simulink library "WECSim_Lib_Body_Elements"  (R2020b)
settings: Solver=VariableStepAuto  StartTime=0.0  StopTime=10.0  RelTol=1e-3
undefined symbols (not defined in the file or in its folder): body, simu, waves, X, Y, Z
libraries: nesl_utility x22, sm_lib x16, $bdroot x9, vrlib x3
(part 1 of 5)
settings Model: Creator=kmruehl  LastModifiedBy=rsaucie
settings ConfigComp: CovBoundaryAbsTol=1.0e-5

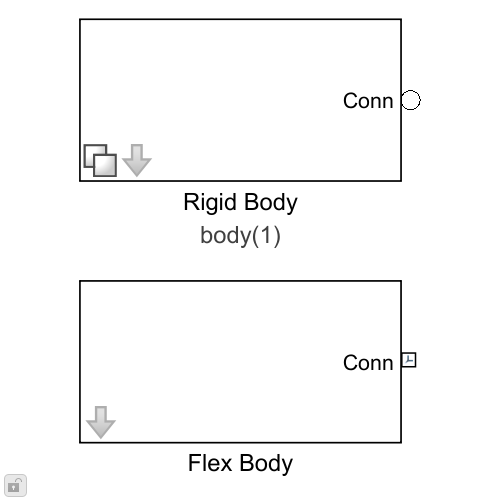
[thumbnail: Simulink's stored preview of the top-level diagram]
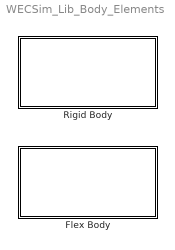
== system WECSim_Lib_Body_Elements ==
  Flex Body : Subsystem  VariantControl=(default)  mask(Flex Body){body=body(1)}
      mask prompts: body "Body Number:"
      mask help:
      | A Flex Body may contain generalized body modes that account for various bending, shear or other deformation modes. The BEM output must contain data for these additional DOFs.
      |
      | The variable name input below must be 'body(i)' where i=1,2,...
      | body(i) must be defined in the input file with the following fields:
      |
      |     .flexHydroBody = 1 (required)
      |             Float.
      |             Flag that creates a flex body. Set equal to 1 if the BEM data contains more than 6 degrees of freedom.
      |     .filename (required)
      |             String.
      |             The file path specifying the .h5 file for the body.
      |     .mass (required)
      |             Float or string.
      |             The translational interia or mass of the body in kg. If a string, the value must be 'equilibrium'. Default = [ ]
      |     .momOfIntertia (required)
      |             3x1 vector [Ixx Iyy Izz].
      |             Rotational intertia of the body in kg*m^2. Default = [ ]
      |     .geometryFile (optional)
      |             String
      |             Path to the geometry file of the body (.stl). Required for nonlinear hydrodynamics or visualization. Default = [ ]
      mask init:
      | if exist('body','var')
      |     % geometry file name
      |     h=[gcb '/Structure/Body Properties'];
      |     geomFile=body.geometryFile;
      |     set_param(h,'ExtGeomFileName',geomFile);
      |     geomType='STL';
      |     % split version e.g. '9.10.0.16028 (R2021a)' into 9, 10, 0, NaN.
      |     % cannot compare str2double('9.10') because it becomes '9.1' 
      |     ver=split(version,'.');
      |     ver=str2double(ver(1:3));
      |     if ver(1) < 9 || (ver(1) == 9 && ver(2) < 6)
      |        set_param(h,'ExtGeomFileType',geomType);
      |     end
      |     % toWorkSpace: outputs
      |     h=[gcb '/To Workspace'];
      |     responseName=['body' num2str(body.number) '_out'];
      |     set_param(h,'VariableName',responseName);
      |     % toWorkSpace: hydrostatic pressures
      |     h=[gcb '/Hydrostatic Restoring Force Calculation/Hydrostatic Restoring Force Calculation/Linear and Nonlinear Restoring Force Variant Subsystem/Nonlinear Hydrostatic Restoring Force/To Workspace1'];
      |     responseName=['body' num2str(body.number) '_hspressure_out'];
      |     set_param(h,'VariableName',responseName); 
      |     % toWorkSpace: wave pressures (nonlinear Froude-Krylov)
      |     h=[gcb '/Wave Diffraction and Excitation Force Calculation/Wave Diffraction and Excitation Force Calculation/Nonlinear FK Force Variant Subsystem/With Nonlinear FroudeKrylov Force/To Workspace'];
      |     responseName=['body' num2str(body.number) '_wavenonlinearpressure_out'];
      |     set_param(h,'VariableName',responseName);
      |     % toWorkSpace: wave pressures (linear Froude-Krylov)
      |     h=[gcb '/Wave Diffraction and Excitation Force Calculation/Wave Diffraction and Excitation Force Calculation/Nonlinear FK Force Variant Subsystem/With Nonlinear FroudeKrylov Force/To Workspace1'];
      |     responseName=['body' num2str(body.number) '_wavelinearpressure_out'];
      |     set_param(h,'VariableName',responseName);
      |     % position: GoTo 
      |     h=[gcb '/Goto'];
      |     responseName=['disp' num2str(body.number)];
      |     set_param(h,'GotoTag',responseName);
      |     % position: From
      |     h=[gcb '/From'];
      |     responseName=['disp' num2str(body.number)];
      |     set_param(h,'GotoTag',responseName);
      |     % velocity: GoTo 
      |     h=[gcb '/Goto1'];
      |     responseName=['vel' num2str(body.number)];
      |     set_param(h,'GotoTag',responseName);
      |     % velocity: From 
      |     h=[gcb '/From1'];
      |     responseName=['vel' num2str(body.number)];
      |     set_param(h,'GotoTag',responseName);
      |     % acceleration: GoTo 
      |     h=[gcb '/Goto2'];
      |     responseName=['acc' num2str(body.number)];
      |     set_param(h,'GotoTag',responseName);
      |     % acceleration: From 
      |     h=[gcb '/From2'];
      |     responseName=['acc' num2str(body.number)];
      |     set_param(h,'GotoTag',responseName);
      |     %% Variable Hydro:
      |     % Variant subsystem
      |     h = [gcb '/Variable Hydrodynamics Control/Variable Hydrodynamics Subsystem'];
      |     responseName = ['sv_b' num2str(body.number) '_variableHydro'];
      |     set_param(h,'VariantControl',responseName);
      |     % body_hydroForceIndex To Workspace tags
      |     h=[gcb '/Variable Hydrodynamics Control/Variable Hydrodynamics Subsystem/variableHydro/To Workspace'];
      |     responseName=['body' num2str(body.number) '_hydroForceIndex'];
      |     set_param(h,'VariableName',responseName); 
      |     % body_hydroForceIndex From tags
      |     h=[gcb '/Variable Hydrodynamics Control/Variable Hydrodynamics Subsystem/variableHydro/From'];
      |     responseName=['body' num2str(body.number) '_hydroForceIndex'];
      |     set_param(h,'GotoTag',responseName);
      |     % body_hydroForce GoTo
      |     h=[gcb '/Variable Hydrodynamics Control/Goto'];
      |     responseName=['body' num2str(body.number) '_hydroForce'];
      |     set_param(h,'GotoTag',responseName);
      |     % body_hydroForce From tags
      |     h=[gcb '/Wave Diffraction and Excitation Force Calculation/Wave Diffraction and Excitation Force Calculation/From'];
      |     responseName=['body' num2str(body.number) '_hydroForce'];
      |     set_param(h,'GotoTag',responseName);
      |     h=[gcb '/Wave Radiation Forces Calculation/Wave Radiation Forces Calculation/From'];
      |     responseName=['body' num2str(body.number) '_hydroForce'];
      |     set_param(h,'GotoTag',responseName);
      |     h=[gcb '/Wave Radiation Forces Calculation/Wave Radiation Forces Calculation/SS CI and Constant-Damping-CoeVariant Subsystem/Constant Coefficients/From'];
      |     responseName=['body' num2str(body.number) '_hydroForce'];
      |     set_param(h,'GotoTag',responseName);
      |     h=[gcb '/Wave Radiation Forces Calculation/Wave Radiation Forces Calculation/SS CI and Constant-Damping-CoeVariant Subsystem/Convolution Integral Calculation/Convolution Variant Subsystem/Convolution Integral Calculation/From'];
      |     responseName=['body' num2str(body.number) '_hydroForce'];
      |     set_param(h,'GotoTag',responseName);
      |     h=[gcb '/Wave Radiation Forces Calculation/Wave Radiation Forces Calculation/SS CI and Constant-Damping-CoeVariant Subsystem/Convolution Integral Calculation/Convolution Variant Subsystem/Convolution Integral Surface Calculation/From'];
      |     responseName=['body' num2str(body.number) '_hydroForce'];
      |     set_param(h,'GotoTag',responseName);
      |     h=[gcb '/Hydrostatic Restoring Force Calculation/Hydrostatic Restoring Force Calculation/Linear and Nonlinear Restoring Force Variant Subsystem/Linear Hydrostatic Restoring Force/From'];
      |     responseName=['body' num2str(body.number) '_hydroForce'];
      |     set_param(h,'GotoTag',responseName);
      |     h=[gcb '/Hydrostatic Restoring Force Calculation/Hydrostatic Restoring Force Calculation/Linear and Nonlinear Restoring Force Variant Subsystem/Nonlinear Hydrostatic Restoring Force/From'];
      |     responseName=['body' num2str(body.number) '_hydroForce'];
      |     set_param(h,'GotoTag',responseName);
      |     h=[gcb '/Hydrostatic Restoring Force Calculation/Hydrostatic Restoring Force Calculation/From'];
      |     responseName=['body' num2str(body.number) '_hydroForce'];
      |     set_param(h,'GotoTag',responseName);
      |     h=[gcb '/Morrison Element and Viscous Damping Force Calculation/From'];
      |     responseName=['body' num2str(body.number) '_hydroForce'];
      |     set_param(h,'GotoTag',responseName);
      |     h=[gcb '/Additional Linear Damping Force Calculation/From'];
      |     responseName=['body' num2str(body.number) '_hydroForce'];
      |     set_param(h,'GotoTag',responseName);
      |     h=[gcb '/FlexibleBody/From'];
      |     responseName=['body' num2str(body.number) '_hydroForce'];
      |     set_param(h,'GotoTag',responseName);
      |     % Update body.hydroForce constant data type
      |     h=[gcb '/Variable Hydrodynamics Control/Constant'];
      |     busName=['Bus: bus_body' num2str(body.number) '_hydroForce'];
      |     set_param(h,'OutDataTypeStr',busName);
      |     %%
      |     % Flex Body Morison Element: Off
      |     h = [gcb '/Morrison Element and Viscous Damping Force Calculation/Morison Element and Viscous Damping Force Calculation/Morison Element Variant Subsystem/Morison Element Off'];
      |     responseName = ['sv_b' num2str(body.number) '_MEOff'];
      |     set_param(h,'VariantControl',responseName);
      |     %%
      |     % Flex Body Morison Element: On
      |     h = [gcb '/Morrison Element and Viscous Damping Force Calculation/Morison Element and Viscous Damping Force Calculation/Morison Element Variant Subsystem/Morison Element On'];
      |     responseName = ['sv_b' num2str(body.number) '_MEOn'];
      |     set_param(h,'VariantControl',responseName);
      |     %%
      |     % Flex Body Nonlinear FroudeKrylov Force: Off
      |     h = [gcb '/Wave Diffraction and Excitation Force Calculation/Wave Diffraction and Excitation Force Calculation/Nonlinear FK Force Variant Subsystem/No Nonlinear FroudeKrylov Force'];
      |     responseName = ['sv_b' num2str(body.number) '_linearHydro'];
      |     set_param(h,'VariantControl',responseName);
      |     %%
      |     % Flex Body Nonlinear FroudeKrylov Force: On
      |     h = [gcb '/Wave Diffraction and Excitation Force Calculation/Wave Diffraction and Excitation Force Calculation/Nonlinear FK Force Variant Subsystem/With Nonlinear FroudeKrylov Force'];
      |     responseName = ['sv_b' num2str(body.number) '_nonlinearHydro'];
      |     set_param(h,'VariantControl',responseName);
      |     %%
      |     % Flex Body Nonlinear Restoring: Off
      |     h = [gcb '/Hydrostatic Restoring Force Calculation/Hydrostatic Restoring Force Calculation/Linear and Nonlinear Restoring Force Variant Subsystem/Linear Hydrostatic Restoring Force'];
      |     responseName = ['sv_b' num2str(body.number) '_linearHydro'];
      |     set_param(h,'VariantControl',responseName);
      |     %%
      |     % Flex Body Nonlinear Restoring: On
      |     h = [gcb '/Hydrostatic Restoring Force Calculation/Hydrostatic Restoring Force Calculation/Linear and Nonlinear Restoring Force Variant Subsystem/Nonlinear Hydrostatic Restoring Force'];
      |     responseName = ['sv_b' num2str(body.number) '_nonlinearHydro'];
      |     set_param(h,'VariantControl',responseName);
      |     %%
      |     % Flex Body Nonlinear FroudeKrylov or Restoring: Instantaneous Free Surface
      |     h = [gcb '/Nonlinear Wave Elevation/Linear or Instantaneous Free Surface/Instantaneous Water Free Surface'];
      |     responseName = ['sv_b' num2str(body.number) '_instFS'];
      |     set_param(h,'VariantControl',responseName);
      |     %%
      |     % Flex Body Nonlinear FroudeKrylov or Restoring: Mean Free Surface
      |     h = [gcb '/Nonlinear Wave Elevation/Linear or Instantaneous Free Surface/Mean Water Free Surface'];
      |     responseName = ['sv_b' num2str(body.number) '_meanFS'];
      |     set_param(h,'VariantControl',responseName);
      |     %%
      | end
      mask Help:
      | A Flex Body may contain generalized body modes that account for various bending, shear or other deformation modes. The BEM output must contain data for these additional DOFs.
      | 
      | The variable name input below must be 'body(i)' where i=1,2,...
      | body(i) must be defined in the input file with the following fields:
      | 
      |     .flexHydroBody = 1 (required)
      |             Float.
      |             Flag that creates a flex body. Set equal to 1 if the BEM data contains more than 6 degrees of freedom.
      |     .filename (required)
      |             String.
      |             The file path specifying the .h5 file for the body.
      |     .mass (required)
      |             Float or string.
      |             The translational interia or mass of the body in kg. If a string, the value must be 'equilibrium'. Default = [ ]
      |     .momOfIntertia (required)
      |             3x1 vector [Ixx Iyy Izz].
      |             Rotational intertia of the body in kg*m^2. Default = [ ]
      |     .geometryFile (optional)
      |             String
      |             Path to the geometry file of the body (.stl). Required for nonlinear hydrodynamics or visualization. Default = [ ]
  Rigid Body : Subsystem  Variant=on  AllowZeroVariantControls=on  mask(Rigid Body){body=body(1)}
      mask prompts: body "Body Number:"
      mask help:
      | A rigid body has no generalized body modes. It can be a standard hydrodynamic body, a drag body, or a non-hydrodynamic body.
      |
      | The variable name input below must be 'body(i)' where i=1,2,...
      | body(i) must be defined in the input file with the fields appropriate to each variant.
      mask init:
      | if exist('body','var')
      |     %%
      |     % Hydro Body
      |     h = [gcb '/Hydrodynamic Body'];
      |     responseName = ['sv_b' num2str(body.number) '_hydroBody'];
      |     set_param(h,'VariantControl',responseName);
      |     %%
      |     % Hydro Body Morison Element: Off
      |     h = [gcb '/Hydrodynamic Body/Morison Element and Viscous Damping Force Calculation/Morison Element Variant Subsystem/Morison Element Off'];
      |     responseName = ['sv_b' num2str(body.number) '_MEOff'];
      |     set_param(h,'VariantControl',responseName);
      |     %%
      |     % Hydro Body Morison Element: On
      |     h = [gcb '/Hydrodynamic Body/Morison Element and Viscous Damping Force Calculation/Morison Element Variant Subsystem/Morison Element On'];
      |     responseName = ['sv_b' num2str(body.number) '_MEOn'];
      |     set_param(h,'VariantControl',responseName);
      |     %%
      |     % Hydro Body Nonlinear Froude Krylov Force: Off
      |     h = [gcb '/Hydrodynamic Body/Wave Diffraction and Excitation Force Calculation/Nonlinear FK Force Variant Subsystem/No Nonlinear FroudeKrylov Force'];
      |     responseName = ['sv_b' num2str(body.number) '_linearHydro'];
      |     set_param(h,'VariantControl',responseName);
      |     %%
      |     % Hydro Body Nonlinear Froude Krylov Force: On
      |     h = [gcb '/Hydrodynamic Body/Wave Diffraction and Excitation Force Calculation/Nonlinear FK Force Variant Subsystem/With Nonlinear FroudeKrylov Force'];
      |     responseName = ['sv_b' num2str(body.number) '_nonlinearHydro'];
      |     set_param(h,'VariantControl',responseName);
      |     %%
      |     % Hydro Body Nonlinear Restoring: Off
      |     h = [gcb '/Hydrodynamic Body/Hydrostatic Restoring Force Calculation/Linear and Nonlinear Restoring Force Variant Subsystem/Linear Hydrostatic Restoring Force'];
      |     responseName = ['sv_b' num2str(body.number) '_linearHydro'];
      |     set_param(h,'VariantControl',responseName);
      |     %%
      |     % Hydro Body Nonlinear Restoring: On
      |     h = [gcb '/Hydrodynamic Body/Hydrostatic Restoring Force Calculation/Linear and Nonlinear Restoring Force Variant Subsystem/Nonlinear Hydrostatic Restoring Force'];
      |     responseName = ['sv_b' num2str(body.number) '_nonlinearHydro'];
      |     set_param(h,'VariantControl',responseName);
      |     %%
      |     % Hydro Body Regular Excitation Passive Yaw: Off
      |     h = [gcb '/Hydrodynamic Body/Wave Diffraction and Excitation Force Calculation/Linear Wave Excitation Force Variant Subsystem/Regular Wave ' newline 'Excitation Force'];
      |     responseName = ['sv_regularWaves_b' num2str(body.number)];
      |     set_param(h,'VariantControl',responseName);
      |     %%
      |     % Hydro Body Regular Excitation Passive Yaw: On
      |     h = [gcb '/Hydrodynamic Body/Wave Diffraction and Excitation Force Calculation/Linear Wave Excitation Force Variant Subsystem/Regular Wave ' newline 'NonLinear Yaw'];
      |     responseName = ['sv_regularWavesYaw_b' num2str(body.number)];
      |     set_param(h,'VariantControl',responseName);
      |     %%    
      |     % Hydro Body Irregular Excitation Passive Yaw: Off
      |     h = [gcb '/Hydrodynamic Body/Wave Diffraction and Excitation Force Calculation/Linear Wave Excitation Force Variant Subsystem/Irregular Wave ' newline 'Excitation Force'];
      |     responseName = ['sv_irregularWaves_b' num2str(body.number)];
      |     set_param(h,'VariantControl',responseName);
      |     %%
      |     % Hydro Body Irregular Excitation Passive Yaw: On
      |     h = [gcb '/Hydrodynamic Body/Wave Diffraction and Excitation Force Calculation/Linear Wave Excitation Force Variant Subsystem/Irregular Wave ' newline 'NonLinearYaw'];
      |     responseName = ['sv_irregularWavesYaw_b' num2str(body.number)];
      |     set_param(h,'VariantControl',responseName);
      |     %%
      |     % Hydro Body Nonlinear Froude Krylov or Restoring: Instantaneous Free Surface
      |     h = [gcb '/Hydrodynamic Body/Nonlinear Wave Elevation/Linear or Instantaneous Free Surface/Instantaneous Water Free Surface'];
      |     responseName = ['sv_b' num2str(body.number) '_instFS'];
      |     set_param(h,'VariantControl',responseName);
      |     %%
      |     % Hydro Body Nonlinear Froude Krylov or Restoring: Mean Free Surface
      |     h = [gcb '/Hydrodynamic Body/Nonlinear Wave Elevation/Linear or Instantaneous Free Surface/Mean Water Free Surface'];
      |     responseName = ['sv_b' num2str(body.number) '_meanFS'];
      |     set_param(h,'VariantControl',responseName);
      |     %% Variable hydro on/off
      |     % Variable hydro control - variable hydro off
      |     h = [gcb '/Hydrodynamic Body/Variable Hydrodynamics Control/Variable Hydrodynamics Subsystem/noVariableHydro'];
      |     responseName = ['sv_b' num2str(body.number) '_noVariableHydro'];
      |     set_param(h,'VariantControl',responseName);
      |     % Variable hydro control - variable hydro on
      |     h = [gcb '/Hydrodynamic Body/Variable Hydrodynamics Control/Variable Hydrodynamics Subsystem/variableHydro'];
      |     responseName = ['sv_b' num2str(body.number) '_variableHydro'];
      |     set_param(h,'VariantControl',responseName);
      |     % CIC - variable hydro off
      |     h = [gcb '/Hydrodynamic Body/Wave Radiation Forces Calculation/SS CI and Constant-Damping-CoeVariant Subsystem/Convolution Integral Calculation/Convolution Variant Subsystem/Convolution Integral Calculation'];
      |     responseName = ['sv_b' num2str(body.number) '_noVariableHydro'];
      |     set_param(h,'VariantControl',responseName);
      |     % CIC - variable hydro on
      |     h = [gcb '/Hydrodynamic Body/Wave Radiation Forces Calculation/SS CI and Constant-Damping-CoeVariant Subsystem/Convolution Integral Calculation/Convolution Variant Subsystem/Convolution Integral Surface Calculation'];
      |     responseName = ['sv_b' num2str(body.number) '_variableHydro'];
      |     set_param(h,'VariantControl',responseName);
      |     %%
      |     % Drag Body
      |     h = [gcb '/Drag Body'];
      |     responseName = ['sv_b' num2str(body.number) '_dragBody'];
      |     set_param(h,'VariantControl',responseName);
      |     %%
      |     % Drag Body Morison Element: Off
      |     h = [gcb '/Drag Body/Morison Element and Viscous Damping Force Calculation/Morison Element Variant Subsystem/Morison Element Off'];
      |     responseName = ['sv_b' num2str(body.number) '_MEOff'];
      |     set_param(h,'VariantControl',responseName);
      |     %%
      |     % Drag Body Morison Element: On
      |     h = [gcb '/Drag Body/Morison Element and Viscous Damping Force Calculation/Morison Element Variant Subsystem/Morison Element On'];
      |     responseName = ['sv_b' num2str(body.number) '_MEOn'];
      |     set_param(h,'VariantControl',responseName);
      |     %% 
      |     % Hydro Body QTF: Off
      |     h = [gcb '/Hydrodynamic Body/Wave Diffraction and Excitation Force Calculation/Second Order Excitation Force Variant Subsystem/No Second Order Excitation Force'];
      |     responseName = ['sv_b' num2str(body.number) '_noSecondOrderExt'];
      |     set_param(h,'VariantControl',responseName);
      |     %%
      |     % Hydro Body QTF: On
      |     h = [gcb '/Hydrodynamic Body/Wave Diffraction and Excitation Force Calculation/Second Order Excitation Force Variant Subsystem/With Second Order Excitation Force'];
      |     responseName = ['sv_b' num2str(body.number) '_secondOrderExt'];
      |     set_param(h,'VariantControl',responseName);
      |     %%
      |     % Set zero active variant controls to prevent label issue
      |     set_param(gcb,'AllowZeroVariantControls','on');
      | end
      | clear bc h geomFile responseName
      settings: AttributesFormatString=%<body>
      mask Help:
      | A rigid body has no generalized body modes. It can be a standard hydrodynamic body, a drag body, or a non-hydrodynamic body.
      | 
      | The variable name input below must be 'body(i)' where i=1,2,...
      | body(i) must be defined in the input file with the fields appropriate to each variant.

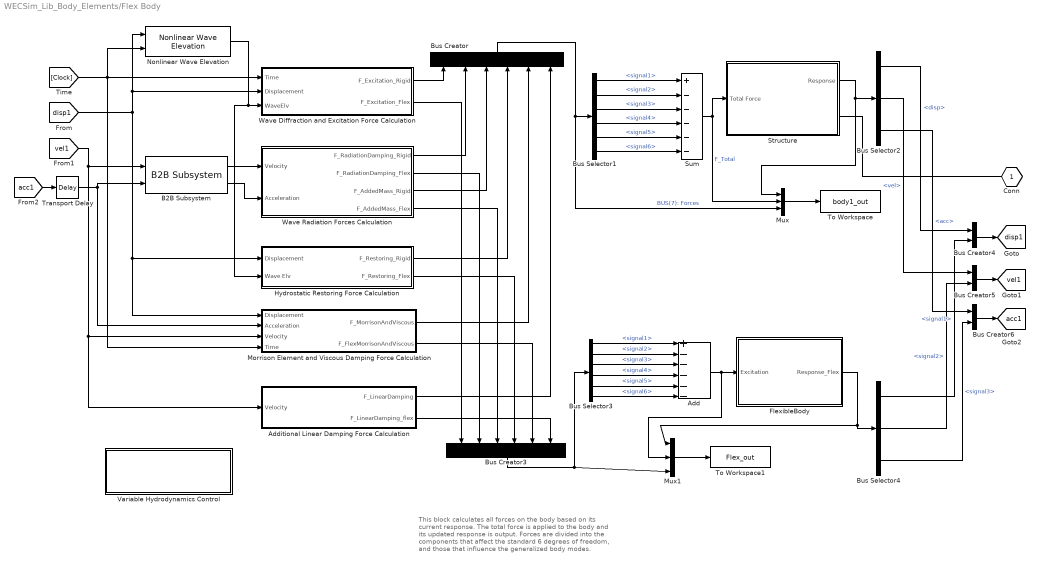
== system WECSim_Lib_Body_Elements/Flex Body ==
  note: This block calculates all forces on the body based on its current response. The total force is applied to the body and its updated response is output.
      |
      | Forces are divided into the components that affect the standard 6 degrees of freedom, and those that influence the generalized body modes.
  Add : Sum  Inputs=+-----
  Additional Linear Damping Force Calculation : Subsystem
  B2B Subsystem : $bdroot/Rigid Body/Hydrodynamic Body/B2B Subsystem  SystemSampleTime=-1  VariantActivationTime=update diagram  EmptyChoice=off  PassThrough=off  PassThroughVariantControl=(default)  EmptyChoiceVariantControl=(default)  Latency=0  AutoFrameSizeCalculation=off
  Bus Creator : BusCreator  Inputs=6
  Bus Creator3 : BusCreator  Inputs=6
  Bus Creator4 : BusCreator  Inputs=2
  Bus Creator5 : BusCreator  Inputs=2
  Bus Creator6 : BusCreator  Inputs=2
  Bus Selector1 : BusSelector  OutputSignals=signal1,signal2,signal3,signal4,signal5,signal6
  Bus Selector2 : BusSelector  OutputSignals=disp,vel,acc
  Bus Selector3 : BusSelector  OutputSignals=signal1,signal2,signal3,signal4,signal5,signal6
  Bus Selector4 : BusSelector  OutputSignals=signal1,signal2,signal3
  FlexibleBody : Subsystem
  Hydrostatic Restoring Force Calculation : Subsystem
  Morrison Element and Viscous Damping Force Calculation : Subsystem
  Mux : Mux  Inputs=3
  Mux1 : Mux  Inputs=3
  Nonlinear Wave Elevation : $bdroot/Rigid Body/Hydrodynamic Body/Nonlinear Wave Elevation  SystemSampleTime=simu.nonlinearDt  VariantActivationTime=update diagram  EmptyChoice=off  PassThrough=off  PassThroughVariantControl=(default)  EmptyChoiceVariantControl=(default)  Latency=0  AutoFrameSizeCalculation=off
  Structure : Subsystem
  Sum : Sum  Inputs=+-----
  To Workspace : ToWorkspace  VariableName=body1_out  SaveFormat=Structure With Time  SampleTime=simu.dtOut
  To Workspace1 : ToWorkspace  VariableName=Flex_out  SaveFormat=Structure With Time  SampleTime=simu.dtOut
  Transport Delay : TransportDelay  DelayTime=10e-8
  Variable Hydrodynamics Control : Subsystem  mask{body=body}
      mask prompts: body "Body Name:"
  Wave Diffraction and Excitation Force Calculation : Subsystem
  Wave Radiation Forces Calculation : Subsystem
  Conn : PMIOPort  Side=Right
  tag scope: acc1=global, disp1=global, vel1=global
  wires:
  Transport Delay/1 -> Morrison Element and Viscous Damping Force Calculation/2(Acceleration), B2B Subsystem/2
  [acc1] -> Transport Delay/1
  Morrison Element and Viscous Damping Force Calculation/1(F_MorrisonAndViscous) -> Bus Creator/5
  Hydrostatic Restoring Force Calculation/2(F_Restoring_Flex) -> Bus Creator3/4
  Bus Selector2/3 -> Bus Creator6/1  "<acc>"
  Bus Selector2/2 -> Bus Creator5/1  "<vel>"
  Bus Creator6/1 -> [acc1]
  Bus Creator5/1 -> [vel1]
  Bus Creator4/1 -> [disp1]
  Bus Selector2/1 -> Bus Creator4/1  "<disp>"
  Bus Selector3/6 -> Add/6  "<signal6>"
  Additional Linear Damping Force Calculation/2(F_LinearDamping_flex) -> Bus Creator3/6
  Bus Selector3/5 -> Add/5  "<signal5>"
  Morrison Element and Viscous Damping Force Calculation/2("F_FlexMorrisonAndViscous ") -> Bus Creator3/5
  Additional Linear Damping Force Calculation/1(F_LinearDamping) -> Bus Creator/6
  Bus Selector4/3 -> Bus Creator6/2  "<signal3>"
  Bus Selector4/2 -> Bus Creator5/2  "<signal2>"
  Bus Selector4/1 -> Bus Creator4/2  "<signal1>"
  FlexibleBody/1(Response_Flex) -> Mux1/1, Bus Selector4/1
  Add/1 -> FlexibleBody/1(Excitation), Mux1/2
  Bus Selector3/4 -> Add/4  "<signal4>"
  Bus Selector3/3 -> Add/3  "<signal3>"
  Bus Selector3/2 -> Add/2  "<signal2>"
  Bus Selector3/1 -> Add/1  "<signal1>"
  Bus Creator3/1 -> Mux1/3, Bus Selector3/1
  Wave Radiation Forces Calculation/4(F_AddedMass_Flex) -> Bus Creator3/3
  Wave Radiation Forces Calculation/2(F_RadiationDamping_Flex) -> Bus Creator3/2
  Wave Diffraction and Excitation Force Calculation/2(F_Excitation_Flex) -> Bus Creator3/1
  Mux1/1 -> To Workspace1/1
  [Clock] -> Wave Diffraction and Excitation Force Calculation/1(Time), Morrison Element and Viscous Damping Force Calculation/4(Time), Nonlinear Wave Elevation/2
  Wave Radiation Forces Calculation/3(F_AddedMass_Rigid) -> Bus Creator/3
  Wave Diffraction and Excitation Force Calculation/1(F_Excitation_Rigid) -> Bus Creator/1
  Wave Radiation Forces Calculation/1(F_RadiationDamping_Rigid) -> Bus Creator/2
  Hydrostatic Restoring Force Calculation/1(F_Restoring_Rigid) -> Bus Creator/4
  Nonlinear Wave Elevation/1 -> Wave Diffraction and Excitation Force Calculation/3(WaveElv), Hydrostatic Restoring Force Calculation/2(Wave Elv)
  [disp1] -> Hydrostatic Restoring Force Calculation/1(Displacement), Morrison Element and Viscous Damping Force Calculation/1(Displacement), Wave Diffraction and Excitation Force Calculation/2(Displacement), Nonlinear Wave Elevation/1
  B2B Subsystem/1 -> Wave Radiation Forces Calculation/1(Velocity)
  B2B Subsystem/2 -> Wave Radiation Forces Calculation/2(Acceleration)
  [vel1] -> B2B Subsystem/1, Morrison Element and Viscous Damping Force Calculation/3(Velocity), Additional Linear Damping Force Calculation/1(Velocity)
  Bus Selector1/6 -> Sum/6  "<signal6>"
  Bus Selector1/1 -> Sum/1  "<signal1>"
  Bus Selector1/2 -> Sum/2  "<signal2>"
  Bus Selector1/5 -> Sum/5  "<signal5>"
  Bus Selector1/3 -> Sum/3  "<signal3>"
  Bus Selector1/4 -> Sum/4  "<signal4>"
  Mux/1 -> To Workspace/1
  Sum/1 -> Structure/1(Total Force), Mux/2  "F_Total"
  Structure/1(Response) -> Bus Selector2/1, Mux/1
  Bus Creator/1 -> Bus Selector1/1, Mux/3  "BUS(7): Forces"
  connections:
  Conn/RConn1 -- Structure/RConn1

== system WECSim_Lib_Body_Elements/Rigid Body ==
  note: 1) Add Subsystem or Model blocks as valid variant choices.
      | 2) You cannot connect blocks at this level. At simulation, connectivity is automatically
      | determined, based on the active variant and port name matching.
  Drag Body : Subsystem  VariantControl=sv_b1_dragBody  mask(Drag Body){body=body}
      mask prompts: body "Body Name:"
      mask help:
      | A drag body contains six degrees of freedom in x, y, z and Mx, My, Mz. It contains a buoyant force, linear damping force, and Morison Element and viscous forces. It is not influenced by wave excitation, radiation damping or radiation added mass.
      |
      | The variable name input below must be 'body(i)' where i=1,2,...
      | body(i) must be defined in the input file with the following fields:
      |
      |     .mass (required)
      |             Float or string.
      |             The translational interia or mass of the body in kg. If a string, the value must be 'equilibrium'. Default = [ ]
      |     .momOfIntertia (required)
      |             3x1 vector [Ixx Iyy Izz].
      |             Rotational intertia of the body in kg*m^2. Default = [ ]
      |     .filename (required)
      |             String.
      |             The file path specifying the .h5 file for the body.
      |     .name (optional)
      |             String.
      |             Specifies the body name. Default = [ ]
      |     .cg (optional)
      |             3x1 float vector [x y z]
      |     .cb (optional)
      |             3x1 float vector [x y z]
      |             Body center of buoyancy in m. Default = [ ].
      |     .dispVol (optional)
      |             Float.
      |             Displaced volume at the equilibrium position in m^3. Default = [ ]
      |     .geometryFile (optional)
      |             String
      |             Path to the geometry file of the body (.stl). Required for nonlinear hydrodynamics or visualization. Default = [ ]
      mask init:
      | if exist('body','var')
      |     % geometry file name
      |     h=[gcb '/Structure/Body Properties'];
      |     geomFile=body.geometryFile;
      |     set_param(h,'ExtGeomFileName',geomFile);
      |     geomType='STL';
      |     % split version e.g. '9.10.0.16028 (R2021a)' into 9, 10, 0, NaN.
      |     % cannot compare str2double('9.10') because it becomes '9.1' 
      |     ver=split(version,'.');
      |     ver=str2double(ver(1:3));
      |     if ver(1) < 9 || (ver(1) == 9 && ver(2) < 6)
      |        set_param(h,'ExtGeomFileType',geomType);
      |     end
      |     % toWorkSpace: outputs
      |     h=[gcb '/To Workspace'];
      |     responseName=['body' num2str(body.number) '_out'];
      |     set_param(h,'VariableName',responseName);
      |     % position GoTo 
      |     h=[gcb '/Goto'];
      |     responseName=['disp' num2str(body.number)];
      |     set_param(h,'GotoTag',responseName);
      |     % position From
      |     h=[gcb '/From'];
      |     responseName=['disp' num2str(body.number)];
      |     set_param(h,'GotoTag',responseName);
      |     % velocity GoTo 
      |     h=[gcb '/Goto1'];
      |     responseName=['vel' num2str(body.number)];
      |     set_param(h,'GotoTag',responseName);
      |     % velocity From 
      |     h=[gcb '/From1'];
      |     responseName=['vel' num2str(body.number)];
      |     set_param(h,'GotoTag',responseName);
      |     % acceleration GoTo 
      |     h=[gcb '/Goto2'];
      |     responseName=['acc' num2str(body.number)];
      |     set_param(h,'GotoTag',responseName);
      |     % acceleration From 
      |     h=[gcb '/From2'];
      |     responseName=['acc' num2str(body.number)];
      |     set_param(h,'GotoTag',responseName);
      | end
  Hydrodynamic Body : Subsystem  VariantControl=sv_b1_hydroBody  mask(Hydrodynamic Body){body=body}
      mask prompts: body "Body Name:"
      mask help:
      | A Hydrodynamic Body contains six degrees of freedom in x, y, z and Mx, My, Mz. All wave forces interact with a hydrodynamic body.
      |
      | The variable name input below must be 'body(i)' where i=1,2,...
      | body(i) must be defined in the input file with the following fields:
      |
      |     .filename (required)
      |             String.
      |             The file path specifying the .h5 file for the body.
      |     .mass (required)
      |             Float or string.
      |             The translational interia or mass of the body in kg. If a string, the value must be 'equilibrium'. Default = [ ]
      |     .momOfIntertia (required)
      |             3x1 vector [Ixx Iyy Izz].
      |             Rotational intertia of the body in kg*m^2. Default = [ ]
      |     .geometryFile (optional)
      |             String
      |             Path to the geometry file of the body (.stl). Required for nonlinear hydrodynamics or visualization. Default = [ ]
      mask init:
      | if exist('body','var') && ~isempty(body)
      |     % geometry file name
      |     h=[gcb '/Structure/Body Properties'];
      |     geomFile=body.geometryFile;
      |     set_param(h,'ExtGeomFileName',geomFile);
      |     geomType='STL';
      |     % split version e.g. '9.10.0.16028 (R2021a)' into 9, 10, 0, NaN.
      |     % cannot compare str2double('9.10') because it becomes '9.1' 
      |     ver=split(version,'.');
      |     ver=str2double(ver(1:3));
      |     if ver(1) < 9 || (ver(1) == 9 && ver(2) < 6)
      |        set_param(h,'ExtGeomFileType',geomType);
      |     end
      |     % toWorkSpace: outputs
      |     h=[gcb '/To Workspace'];
      |     responseName=['body' num2str(body.number) '_out'];
      |     set_param(h,'VariableName',responseName);
      |     % toWorkSpace: hydrostatic pressures
      |     h=[gcb '/Hydrostatic Restoring Force Calculation/Linear and Nonlinear Restoring Force Variant Subsystem/Nonlinear Hydrostatic Restoring Force/To Workspace1'];
      |     responseName=['body' num2str(body.number) '_hspressure_out'];
      |     set_param(h,'VariableName',responseName); 
      |     % toWorkSpace: wave pressures (non-linear Freude-Krylov)
      |     h=[gcb '/Wave Diffraction and Excitation Force Calculation/Nonlinear FK Force Variant Subsystem/With Nonlinear FroudeKrylov Force/To Workspace'];
      |     responseName=['body' num2str(body.number) '_wavenonlinearpressure_out'];
      |     set_param(h,'VariableName',responseName);
      |     % toWorkSpace: wave pressures (linear Freude-Krylov)
      |     h=[gcb '/Wave Diffraction and Excitation Force Calculation/Nonlinear FK Force Variant Subsystem/With Nonlinear FroudeKrylov Force/To Workspace1'];
      |     responseName=['body' num2str(body.number) '_wavelinearpressure_out'];
      |     set_param(h,'VariableName',responseName);
      | 
      |     % position GoTo 
      |     h=[gcb '/Goto'];
      |     responseName=['disp' num2str(body.number)];
      |     set_param(h,'GotoTag',responseName);
      |     % position From
      |     h=[gcb '/From'];
      |     responseName=['disp' num2str(body.number)];
      |     set_param(h,'GotoTag',responseName);
      | 
      |     % velocity GoTo 
      |     h=[gcb '/Goto1'];
      |     responseName=['vel' num2str(body.number)];
      |     set_param(h,'GotoTag',responseName);
      |     % velocity From 
      |     h=[gcb '/From1'];
      |     responseName=['vel' num2str(body.number)];
      |     set_param(h,'GotoTag',responseName);
      | 
      |     % acceleration GoTo
      |     h=[gcb '/Goto2'];
      |     responseName=['acc' num2str(body.number)];
      |     set_param(h,'GotoTag',responseName);
      |     % acceleration From 
      |     h=[gcb '/From2'];
      |     responseName=['acc' num2str(body.number)];
      |     set_param(h,'GotoTag',responseName);
      | 
      |     % excitation force GoTo
      |     h = [gcb '/Goto3'];
      |     responseName = ['b' num2str(body.number) '_f_excitation'];
      |     set_param(h, 'GotoTag', responseName);
      |     % total force GoTo
      |     h = [gcb '/Goto4'];
      |     responseName = ['b' num2str(body.number) '_f_total'];
      |     set_param(h, 'GotoTag', responseName);
      |     
      |     %% Variable Hydro:
      |     % Variant subsystem
      |     h = [gcb '/Variable Hydrodynamics Control/Variable Hydrodynamics Subsystem'];
      |     responseName = ['sv_b' num2str(body.number) '_variableHydro'];
      |     set_param(h,'VariantControl',responseName);
      |     % body_hydroForceIndex To Workspace tags
      |     h=[gcb '/Variable Hydrodynamics Control/Variable Hydrodynamics Subsystem/variableHydro/To Workspace'];
      |     responseName=['body' num2str(body.number) '_hydroForceIndex'];
      |     set_param(h,'VariableName',responseName); 
      |     % body_hydroForceIndex From tags
      |     h=[gcb '/Variable Hydrodynamics Control/Variable Hydrodynamics Subsystem/variableHydro/From'];
      |     responseName=['body' num2str(body.number) '_hydroForceIndex'];
      |     set_param(h,'GotoTag',responseName);
      |     h=[gcb '/Wave Radiation Forces Calculation/SS CI and Constant-Damping-CoeVariant Subsystem/Convolution Integral Calculation/Convolution Variant Subsystem/Convolution Integral Surface Calculation/From'];
      |     responseName=['body' num2str(body.number) '_hydroForceIndex'];
      |     set_param(h,'GotoTag',responseName);
      |     % body_hydroForce GoTo
      |     h=[gcb '/Variable Hydrodynamics Control/Goto'];
      |     responseName=['body' num2str(body.number) '_hydroForce'];
      |     set_param(h,'GotoTag',responseName);
      |     % body_hydroForce From tags
      |     h=[gcb '/Wave Diffraction and Excitation Force Calculation/From'];
      |     responseName=['body' num2str(body.number) '_hydroForce'];
      |     set_param(h,'GotoTag',responseName);
      |     h=[gcb '/Wave Radiation Forces Calculation/From'];
      |     responseName=['body' num2str(body.number) '_hydroForce'];
      |     set_param(h,'GotoTag',responseName);
      |     h=[gcb '/Wave Radiation Forces Calculation/SS CI and Constant-Damping-CoeVariant Subsystem/Constant Coefficients/From'];
      |     responseName=['body' num2str(body.number) '_hydroForce'];
      |     set_param(h,'GotoTag',responseName);
      |     h=[gcb '/Wave Radiation Forces Calculation/SS CI and Constant-Damping-CoeVariant Subsystem/Convolution Integral Calculation/Convolution Variant Subsystem/Convolution Integral Calculation/From'];
      |     responseName=['body' num2str(body.number) '_hydroForce'];
      |     set_param(h,'GotoTag',responseName);
      |     h=[gcb '/Hydrostatic Restoring Force Calculation/Linear and Nonlinear Restoring Force Variant Subsystem/Linear Hydrostatic Restoring Force/From'];
      |     responseName=['body' num2str(body.number) '_hydroForce'];
      |     set_param(h,'GotoTag',responseName);
      |     h=[gcb '/Hydrostatic Restoring Force Calculation/Linear and Nonlinear Restoring Force Variant Subsystem/Nonlinear Hydrostatic Restoring Force/From'];
      |     responseName=['body' num2str(body.number) '_hydroForce'];
      |     set_param(h,'GotoTag',responseName);
      |     h=[gcb '/Hydrostatic Restoring Force Calculation/From'];
      |     responseName=['body' num2str(body.number) '_hydroForce'];
      |     set_param(h,'GotoTag',responseName);
      |     h=[gcb '/From3'];
      |     responseName=['body' num2str(body.number) '_hydroForce'];
      |     set_param(h,'GotoTag',responseName);
      |     % Update body.hydroForce constant data type
      |     h=[gcb '/Variable Hydrodynamics Control/Constant'];
      |     busName=['Bus: bus_body' num2str(body.number) '_hydroForce'];
      |     set_param(h,'OutDataTypeStr',busName);
      | end
  Conn : PMIOPort  Side=Right

== system WECSim_Lib_Body_Elements/Flex Body/Additional Linear Damping Force Calculation ==
  Velocity : Inport
  Additional Linear Damping Force Calculation1 : $bdroot/Rigid Body/Hydrodynamic Body/Additional Linear Damping Force Calculation  SystemSampleTime=-1  VariantActivationTime=update diagram  EmptyChoice=off  PassThrough=off  PassThroughVariantControl=(default)  EmptyChoiceVariantControl=(default)  Latency=0  AutoFrameSizeCalculation=off
  Bus Selector : BusSelector  OutputSignals=linearDamping
  Selector : Selector  InputPortWidth=body.dof  IndexOptions=Index vector (dialog)  Indices=[1:6]  OutputSizes=1
  Selector1 : Selector  InputPortWidth=body.dof  IndexOptions=Index vector (dialog)  Indices=[7:body.dofEnd]  OutputSizes=1
  F_LinearDamping : Outport  PortDimensions=6
  F_LinearDamping_flex : Outport  Port=2  PortDimensions=body.gbmDOF
  wires:
  [body1_hydroForce] -> Bus Selector/1
  Bus Selector/1 -> Additional Linear Damping Force Calculation1/2  "<linearDamping>"
  Additional Linear Damping Force Calculation1/1 -> Selector1/1, Selector/1
  Velocity/1 -> Additional Linear Damping Force Calculation1/1  "v"
  Selector1/1 -> F_LinearDamping_flex/1
  Selector/1 -> F_LinearDamping/1

== system WECSim_Lib_Body_Elements/Flex Body/FlexibleBody ==
  note: This block solves the governing equations of motion for the flexible degrees of freedom (generalized body modes) using the flex force components. The response of the generalied body modes is output.
  Excitation : Inport
  Add : Sum  Inputs=--+
  Bus Creator : BusCreator  Inputs=3
  Bus Selector : BusSelector  OutputSignals=gbm.mass_ff_inv,gbm.stiffness,gbm.damping,gbm.mass_ff_inv
  GBM : StateSpace  A=body.hydroForce.hf1.gbm.state_space.A  B=body.hydroForce.hf1.gbm.state_space.B  C=body.hydroForce.hf1.gbm.state_space.C  D=body.hydroForce.hf1.gbm.state_space.D  InitialCondition=0
  Mux : Mux  Inputs=2
  Product1 : Product  Multiplication=Matrix(*)
  Product2 : Product  Multiplication=Matrix(*)
  Product4 : Product  Multiplication=Matrix(*)
  acceleration : Product  Multiplication=Matrix(*)
  displacement : Selector  InputPortWidth=body.gbmDOF*2  IndexOptions=Index vector (dialog)  Indices=[1:body.gbmDOF]  OutputSizes=1
  unit matrix : Constant  Value=zeros(body.gbmDOF,1)
  velocity : Selector  InputPortWidth=2*body.gbmDOF  IndexOptions=Index vector (dialog)  Indices=[body.gbmDOF+1:2*body.gbmDOF]  OutputSizes=1
  Response_Flex : Outport
  wires:
  Bus Selector/4 -> Product4/1  "<mass_ff_inv>"
  Bus Selector/3 -> Product2/1  "<damping>"
  Bus Selector/2 -> Product1/1  "<stiffness>"
  Bus Selector/1 -> acceleration/1  "<mass_ff_inv>"
  [body1_hydroForce] -> Bus Selector/1
  acceleration/1 -> Bus Creator/3
  Bus Creator/1 -> Response_Flex/1
  Mux/1 -> GBM/1
  Product4/1 -> Mux/2
  unit matrix/1 -> Mux/1
  Product2/1 -> Add/2
  Add/1 -> acceleration/2
  Product1/1 -> Add/1  "F_AddedMass"
  velocity/1 -> Bus Creator/2, Product2/2
  displacement/1 -> Bus Creator/1, Product1/2
  GBM/1 -> displacement/1, velocity/1
  Excitation/1 -> Add/3, Product4/2

== system WECSim_Lib_Body_Elements/Flex Body/Hydrostatic Restoring Force Calculation ==
  note: Do not link the `Hydrostatic Restoring Force Calculation`
      | to the rigid body block, this will break the Flex Body block.
  Displacement : Inport
  Wave Elv : Inport  Port=2
  Hydrostatic Restoring Force Calculation : Subsystem
  Selector : Selector  InputPortWidth=body.dof  IndexOptions=Index vector (dialog)  Indices=[1:6]  OutputSizes=1
  Selector1 : Selector  InputPortWidth=body.dof  IndexOptions=Index vector (dialog)  Indices=[7:body.dofEnd]  OutputSizes=1
  F_Restoring_Rigid : Outport  PortDimensions=6
  F_Restoring_Flex : Outport  Port=2  PortDimensions=body.gbmDOF
  wires:
  Wave Elv/1 -> Hydrostatic Restoring Force Calculation/2(Wave Elv)
  Displacement/1 -> Hydrostatic Restoring Force Calculation/1(Displacement)  "x"
  Selector1/1 -> F_Restoring_Flex/1
  Selector/1 -> F_Restoring_Rigid/1
  Hydrostatic Restoring Force Calculation/1(F_Restoring) -> Selector/1, Selector1/1  "F_Restoring"

== system WECSim_Lib_Body_Elements/Flex Body/Morrison Element and Viscous Damping Force Calculation ==
  Displacement : Inport
  Acceleration : Inport  Port=2
  Velocity : Inport  Port=3
  Time : Inport  Port=4
  Bus Selector : BusSelector  OutputSignals=quadDrag
  Morison Element and Viscous Damping Force Calculation : $bdroot/Rigid Body/Hydrodynamic Body/Morison Element and Viscous Damping Force Calculation  SystemSampleTime=-1  VariantActivationTime=update diagram  EmptyChoice=off  PassThrough=off  PassThroughVariantControl=(default)  EmptyChoiceVariantControl=(default)  Latency=0  AutoFrameSizeCalculation=off
  Selector : Selector  InputPortWidth=body.dof  IndexOptions=Index vector (dialog)  Indices=[1:6]  OutputSizes=1
  Selector1 : Selector  InputPortWidth=body.dof  IndexOptions=Index vector (dialog)  Indices=[7:body.dofEnd]  OutputSizes=1
  F_MorrisonAndViscous : Outport  PortDimensions=6
  "F_FlexMorrisonAndViscous " : Outport  Port=2  PortDimensions=body.gbmDOF
  wires:
  [body1_hydroForce] -> Bus Selector/1
  Bus Selector/1 -> Morison Element and Viscous Damping Force Calculation/5  "<quadDrag>"
  Selector1/1 -> "F_FlexMorrisonAndViscous "/1
  Selector/1 -> F_MorrisonAndViscous/1
  Morison Element and Viscous Damping Force Calculation/1 -> Selector/1, Selector1/1
  Velocity/1 -> Morison Element and Viscous Damping Force Calculation/3
  Displacement/1 -> Morison Element and Viscous Damping Force Calculation/1
  Time/1 -> Morison Element and Viscous Damping Force Calculation/4
  Acceleration/1 -> Morison Element and Viscous Damping Force Calculation/2

== system WECSim_Lib_Body_Elements/Flex Body/Structure ==
  note: Apply the total force to the body and calculate its response relative to the global reference frame.
      |
      | Output force to apply to another body.
  Total Force : Inport
  Body Properties : sm_lib/Body Elements/File Solid  ExtGeomFileName=geometry/float.stl  UnitType=Custom  ExtGeomFileUnits=m  StepReaderType=HEX  ExportConvexHullGeometry=off  InertiaType=Custom  BasedOnType=Density  Density=1000  DensityUnits=kg/(m^3)  Mass=body.hydroForce.(['hf' num2str(body.variableHydro.hydroForceIndexInitial)]).adjustedMass  MassUnits=kg  CenterOfMass=[0 0 0]  CenterOfMassUnits=m  MomentsOfInertia=body.hydroForce.(['hf' num2str(body.variableHydro.hydroForceIndexInitial)]).adjustedInertia  MomentsOfInertiaUnits=kg*m^2  ProductsOfInertia=body.hydroForce.(['hf' num2str(body.variableHydro.hydroForceIndexInitial)]).adjustedInertiaProducts  ProductsOfInertiaUnits=kg*m^2  GraphicType=FromGeometry  MarkerShape=Sphere  MarkerSize=10  GraphicVisPropType=SimpleVisualProperties  GraphicDiffuseColor=body.viz.color  GraphicOpacity=body.viz.opacity  GraphicSpecularColor=[0.5 0.5 0.5 1.0]  GraphicAmbientColor=[0.15 0.15 0.15 1.0]  GraphicEmissiveColor=[0.0 0.0 0.0 1.0]  GraphicShininess=75  DoExposeReferenceFrame=on  SerializedFrames=<Frames/>
  External Force and Torque : sm_lib/Forces and Torques/External Force and Torque  EnableForceX=off  EnableForceY=off  EnableForceZ=off  EnableForce=on  ForceResolutionFrame=World  EnableTorqueX=off  EnableTorqueY=off  EnableTorqueZ=off  EnableTorque=on  TorqueResolutionFrame=World
  Motion Sensor : $bdroot/Rigid Body/Hydrodynamic Body/Structure/Motion Sensor  SystemSampleTime=-1  VariantActivationTime=update diagram  EmptyChoice=off  PassThrough=off  PassThroughVariantControl=(default)  EmptyChoiceVariantControl=(default)  Latency=0  AutoFrameSizeCalculation=off
  Rigid Transform (Setup CG) : sm_lib/Frames and Transforms/Rigid Transform  RotationMethod=None  FollAlignAxisA=+X  BaseAlignAxisA=+Y  FollAlignAxisB=+Y  BaseAlignAxisB=+Z  RotationStandardAxis=+Y  RotationAngle=0.05  RotationAngleUnits=rad  RotationArbitraryAxis=[0.57735026918962584 0.57735026918962584 0.57735026918962584]  RotationSequenceAxes=FollowerAxes  RotationSequence=XYX  RotationSequenceAngles=[0 0 0]  RotationSequenceAnglesUnits=deg  RotationMatrix=[1 0 0; 0 1 0; 0 0 1]  Quaternion=[1 0 0 0]  TranslationMethod=Cartesian  TranslationCartesianOffset=body.centerGravity  TranslationCartesianOffsetUnits=m  TranslationStandardAxis=+Z  TranslationStandardOffset=0  TranslationStandardOffsetUnits=m  TranslationROffset=0  TranslationROffsetUnits=m  TranslationThetaOffset=0  TranslationThetaOffsetUnits=deg  TranslationZOffset=0  TranslationZOffsetUnits=m
  Rigid Transform (Setup Initial Disp) : sm_lib/Frames and Transforms/Rigid Transform  RotationMethod=ArbitraryAxis  FollAlignAxisA=+X  BaseAlignAxisA=+Y  FollAlignAxisB=+Y  BaseAlignAxisB=+Z  RotationStandardAxis=+Y  RotationAngle=body.initial.angle  RotationAngleUnits=rad  RotationArbitraryAxis=body.initial.axis  RotationSequenceAxes=FollowerAxes  RotationSequence=XYX  RotationSequenceAngles=[0 0 0]  RotationSequenceAnglesUnits=deg  RotationMatrix=[1 0 0; 0 1 0; 0 0 1]  Quaternion=[1 0 0 0]  TranslationMethod=Cartesian  TranslationCartesianOffset=body.initial.displacement  TranslationCartesianOffsetUnits=m  TranslationStandardAxis=+Z  TranslationStandardOffset=0  TranslationStandardOffsetUnits=m  TranslationROffset=0  TranslationROffsetUnits=m  TranslationThetaOffset=0  TranslationThetaOffsetUnits=deg  TranslationZOffset=0  TranslationZOffsetUnits=m
  Selector : Selector  InputPortWidth=6  IndexOptions=Index vector (dialog)  Indices=[1:3]  OutputSizes=1
  Selector1 : Selector  InputPortWidth=6  IndexOptions=Index vector (dialog)  Indices=[4:6]  OutputSizes=1
  Simulink-PS Converter1 : nesl_utility/Simulink-PS Converter  PhysicalDomain=network_engine_domain  SubClassName=ps_input  LeftPortType=input  RightPortType=output  PseudoPeriodic=off  Frequencies=[]  NoiseDistribution=none  NoiseParameters=[]  Unit=1  AffineConversion=off  FilteringAndDerivatives=zero  SimscapeFilterOrder=1  InputFilterTimeConstant=0.001  UdotUserProvided=1
  Simulink-PS Converter2 : nesl_utility/Simulink-PS Converter  PhysicalDomain=network_engine_domain  SubClassName=ps_input  LeftPortType=input  RightPortType=output  PseudoPeriodic=off  Frequencies=[]  NoiseDistribution=none  NoiseParameters=[]  Unit=1  AffineConversion=off  FilteringAndDerivatives=zero  SimscapeFilterOrder=1  InputFilterTimeConstant=0.001  UdotUserProvided=1
  World Frame : sm_lib/Frames and Transforms/World Frame
  Conn Free Surface : PMIOPort  Side=Right
  Response : Outport
  wires:
  Motion Sensor/1 -> Response/1
  Selector1/1 -> Simulink-PS Converter2/1
  Selector/1 -> Simulink-PS Converter1/1
  Total Force/1 -> Selector/1, Selector1/1
  connections:
  Motion Sensor/LConn1 -- World Frame/RConn1
  Rigid Transform (Setup Initial Disp)/LConn1 -- Rigid Transform (Setup CG)/RConn1
  Conn Free Surface/RConn1 -- Rigid Transform (Setup CG)/LConn1
  External Force and Torque/RConn1 -- Motion Sensor/RConn1 -- Body Properties/RConn1 -- Rigid Transform (Setup Initial Disp)/RConn1
  External Force and Torque/LConn2 -- Simulink-PS Converter2/RConn1
  External Force and Torque/LConn1 -- Simulink-PS Converter1/RConn1
